simulink model "pyclops_LQR"  (R2025b)
settings: Solver=ode45  StartTime=0.0  StopTime=10  RelTol=1e-3
values from neighbouring files (symbols this model uses):
  K_lqr = lqr(A0, B0, Q, R)    [func_compute_K_lqr.m]    (also in setup_params.m)
settings Model: Creator=theo  LastModifiedBy=theo

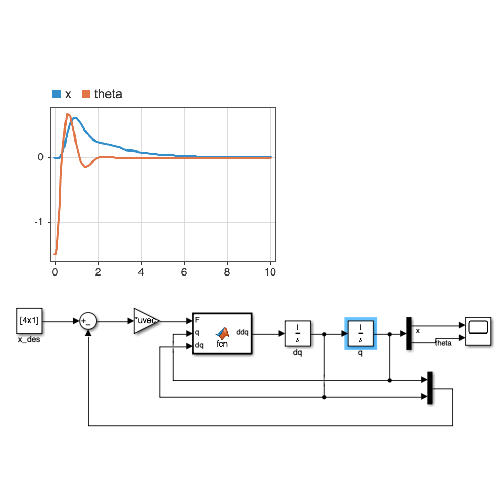
[thumbnail: Simulink's stored preview of the top-level diagram]
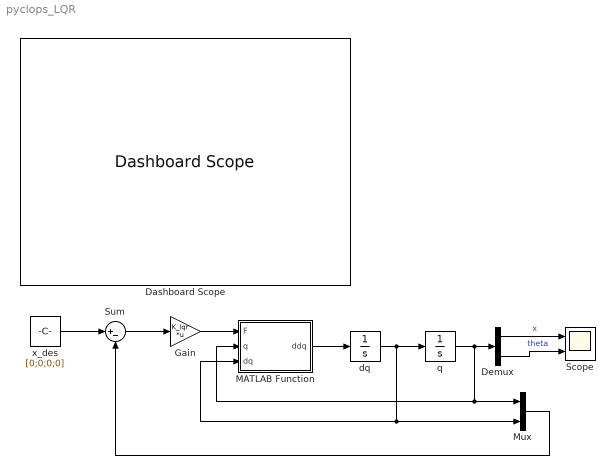
== system pyclops_LQR ==
  Dashboard Scope : DashboardScope  FontColor=[0.0, 0.0, 0.0]
  Demux : Demux  Outputs=2
  Gain : Gain  Gain=K_lqr  Multiplication=Matrix(K*u) (u vector)
  MATLAB Function : MATLAB Function  TreatAsAtomicUnit=on
  Mux : Mux  Inputs=2
  Scope : Scope  NumInputPorts=2
      settings: ActiveDisplayYMinimum=-0.11802529274459451  ActiveDisplayYMaximum=0.062227634701350655
  Sum : Sum  Inputs=|+-
  dq : Integrator  InitialCondition=[0; 0]
  q : Integrator  InitialCondition=[0; -1.5]
  x_des : Constant  Value=[0;0;0;0]
  wires:
  dq/1 -> MATLAB Function/3(dq), Mux/2, q/1
  q/1 -> MATLAB Function/2(q), Mux/1, Demux/1
  MATLAB Function/1(ddq) -> dq/1
  Demux/2 -> Scope/2  "theta"
  Sum/1 -> Gain/1
  Gain/1 -> MATLAB Function/1(F)
  Demux/1 -> Scope/1  "x"
  x_des/1 -> Sum/1
  Mux/1 -> Sum/2

== matlab function pyclops_LQR/MATLAB Function ==
  data: F input; ddq output; q input; dq input
function ddq = fcn(F, q, dq)
%#codegen

    ddq = zeros(2,1);

    % Parameters: [m, M, l, g]
    params = [0.2, 0.5, 0.3, 9.81];

    % Get D, C, G from auto-generated function
    [D, C, G] = func_compute_D_C_G(q, dq, params);

    % Generalized force
    tau = [F; 0];

    % Solve for acceleration
    ddq = D \ (tau - C*dq - G);

end
